simulink model "ConfiguredHevMmVirtualVehicle"  (R2025b)
settings: configuration reference "VehicleVariable" (kept outside this file)
StartFcn:
  | %tic
StopFcn:
  | %toc
model workspace (MAT data in the model file):
  ExtDrvCmdsSwitch = Simulink.Parameter
  ExtDrvCmdsSwitch.Value = 0
  ExtDrvCmdsSwitch.Complexity = 'real'
  ExtDrvCmdsSwitch.Dimensions = [1 1]
  ExtDrvCmdsSwitch.DataType = 'boolean'
  ExtDrvRefSwitch = Simulink.Parameter
  ExtDrvRefSwitch.Value = 0
  ExtDrvRefSwitch.Complexity = 'real'
  ExtDrvRefSwitch.Dimensions = [1 1]
  ExtDrvRefSwitch.DataType = 'boolean'
  ExtEnvSwitch = Simulink.Parameter
  ExtEnvSwitch.Value = 0
  ExtEnvSwitch.Complexity = 'real'
  ExtEnvSwitch.Dimensions = [1 1]
  ExtEnvSwitch.DataType = 'boolean'
  ExtGndSwitch = Simulink.Parameter
  ExtGndSwitch.Value = 0
  ExtGndSwitch.Complexity = 'real'
  ExtGndSwitch.Dimensions = [1 1]
  ExtGndSwitch.DataType = 'boolean'
undefined symbols (not defined in the file or in its folder): AmbTemp, BaroPress, CurvGradRef, CurvRef, DCM, DriverAeroRes, DriverDrivelineRes, DriverInitialGear, DriverPreviewDist, DriverRollRes, DriverShiftTime, DriverTimeConst, DriverTractiveForce, EnvAbsPrs, EnvAirTemp, EnvGrvty, EnvNomFrictionScaling, EnvNominalGrade, EnvScnFrictionMap, EnvScnFrictionMapXBpts, EnvScnFrictionMapYBpts, EnvScnHeightMap, EnvScnHeightMapXBpts, EnvScnHeightMapYBpts, EnvWindVelX, EnvWindVelY, EnvWindVelZ, Gnd, Grade, HazzardCmd, HighBeamCmd, lambda_mux, LeftSignalCmd, LngRef, LowBeamCmd, LtrRef, PhiRef, PlntVehDstCGFrntAxl, PlntVehDstCGRearAxl, PlntVehInitLatPos, PlntVehInitLongPos, PlntVehInitPitchAng, PlntVehInitRollAng, PlntVehInitVertPos, PlntVehInitYawAng, PlntVehMass, PlntVehTrckWdth, PlntVehYawMomentInertia, PlntWhlLdRadiusFrnt, PlntWhlLdRadiusRear, RightSignalCmd, ScnCRRadius, Sim3dSensor, Wind, XRef, YRef, Z
libraries: simulink x28, autolibutils x8, autolibsharedcommon x7, vehdynlibscenariocommon x7, vehdynlibviscommon x4, vehdynlibdriver x2, sim3dgroundtruthsensorlib x2, sim3dlib x2, autolibshared x2, sim3dautolib x2, sl3dlib x1, sharedtransform x1
(part 1 of 6)
settings Model: DataDictionary=VirtualVehicleTemplate.sldd  ModifiedByFormat=The MathWorks, Inc.  SimulationMode=accelerator  ParameterArgumentNames=ExtDrvCmdsSwitch,ExtDrvRefSwitch,ExtEnvSwitch,ExtGndSwitch  Creator=The MathWorks, Inc.  LastModifiedBy=The MathWorks, Inc.
settings ConfigSetRef: SourceName=VehicleVariable

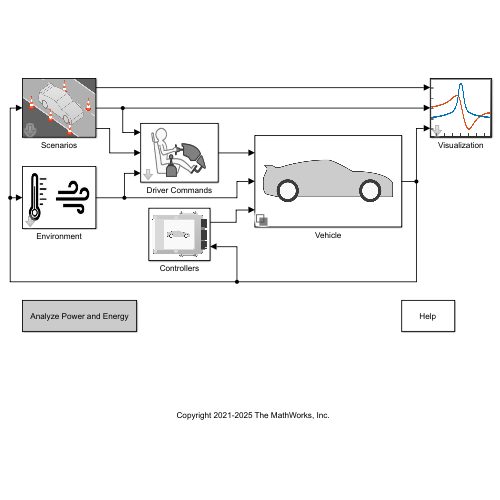
[thumbnail: Simulink's stored preview of the top-level diagram]
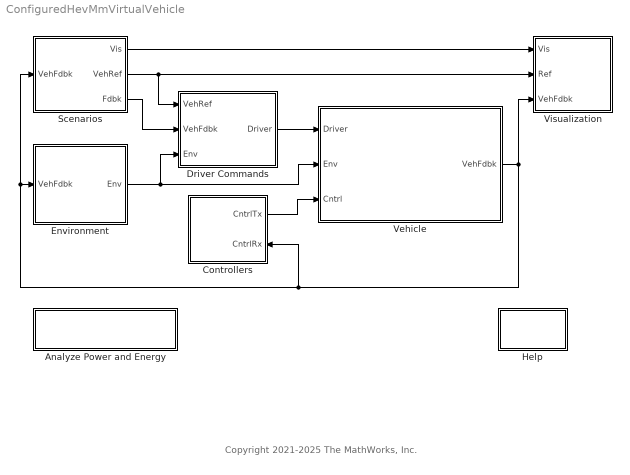
== system ConfiguredHevMmVirtualVehicle ==
  note: Copyright 2021-2025 The MathWorks, Inc.
  Analyze Power and Energy : Subsystem
      settings: OpenFcn=GenerateEnergyReportM2MLX
      mask Display: disp(getString(message('autoblks:autoblkVehMask:powAndEne')))
  Controllers : Subsystem
      settings: PortSchema="{\"entries\":[{\"content\":{\"sides\":[{\"content\":{\"connectorIds\":[]},\"type\":\"ConnectorPlacement.EquallySpacedRectSide\",\"uuid\":\"a925dd9c-6905-4c67-a62c-b22bb69d2bd6\"},{\"content\":{\"connectorIds\":[\"Out1\",\"In1\"],\"side\":\"RIGHT\"},\"type\":\"ConnectorPlacement.EquallySpacedRectSide\",\"uuid\":\"9930ed3e-43a4-46d4-b9ee-7ed64fae32ef\"},{\"content\":{\"connectorIds\":[],\"side\":\"TOP\"},\"type\":\"ConnectorPlacement.EquallySpacedRectSide\",\"uuid\":\"68d2ac4e-de3d-40d3-8b44-059f2a72a6bc\"}]},\"type\":\"ConnectorPlacement.EquallySpacedConnector\",\"uuid\":\"c0be7d07-475b-4046-8bfa-76004f6da9b2\"}],\"packageUris\":[\"http://schema.mathworks.com/mf0/Connector/R2020b\"],\"version\":\"1.0\"}"
      mask Display: image('SystemControllers.png')
  Driver Commands : Subsystem  VariantControl=0  mask(Driver Commands){driverType=Longitudinal Driver}
      mask prompts: driverType "autoblks_reference:autoVirtualRefGen:blkPrm_driverType"
      mask help: autoblks_reference:autoVirtualRefGen:blkDesc_Driver
      mask init:
      | [~]=vdynblksdrvrconfig(gcb);
      mask Help: helpview('autoblks','vvcDriverCommandsHelp')
      mask TypeOptions driverType: autoblks_reference:autoVirtualRefGen:blkCmb_driverType_c1 | autoblks_reference:autoVirtualRefGen:blkCmb_driverType_c2 | autoblks_reference:autoVirtualRefGen:blkCmb_driverType_c3 | autoblks_reference:autoVirtualRefGen:blkCmb_driverType_c4 | autoblks_reference:autoVirtualRefGen:blkCmb_driverType_c5 | autoblks_reference:autoVirtualRefGen:blkCmb_driverType_c6 | autoblks_reference:autoVirtualRefGen:blkCmb_driverType_c7
      mask Callback driverType: [~]=vdynblksdrvrconfig(gcb);
      mask DialogControl driverType Prompt: Vehicle command mode
      mask Display: image('LongitudinalDriver.png');
  Environment : Subsystem  mask(Environment){extEnv=off, extGnd=off}
      mask prompts: extEnv "autoblks_reference:autoVirtualRefGen:blkPrm_extEnv"; extGnd "autoblks_reference:autoVirtualRefGen:blkPrm_extGnd"
      mask help: autoblks_reference:autoVirtualRefGen:blkDesc_Env
      mask Help: helpview('autoblks','vvcEnvironmentHelp')
      mask Callback extEnv: vvcupdateport(gcb,{{'extEnv';'extGnd'},{}},{{'ExtEnv';'ExtGnd'},{}},{{'VVCEnvBUS';'VVCGndSTI4wBUS'},{}});
      mask Callback extGnd: vvcupdateport(gcb,{{'extEnv';'extGnd'},{}},{{'ExtEnv';'ExtGnd'},{}},{{'VVCEnvBUS';'VVCGndSTI4wBUS'},{}});
      mask DialogControl extGroup Prompt: autoblks_reference:autoVirtualRefGen:blkDlg_extGroup
      mask DialogControl extEnv Prompt: Environment
      mask DialogControl extGnd Prompt: Ground
      mask DialogControl EnvButton Prompt: autoblks_reference:autoVirtualRefGen:blkDlg_EnvButton
      mask DialogControl EnvButton Callback: open_system(gcb,'force')
      mask Display: image('Enviroment.png')
  Help : Subsystem
      settings: OpenFcn=helpview('autoblks', 'hybrid_refapp')
      mask Display: disp(getString(message('autoblks:autoblkVehMask:help')))
  Scenarios : Subsystem  mask(Virtual Vehicle Scenario Configuration){extRef=off, extCmd=off}
      mask prompts: extRef "autoblks_reference:autoVirtualRefGen:blkPrm_extRef"; extCmd "autoblks_reference:autoVirtualRefGen:blkPrm_extCmd"
      mask help: autoblks_reference:autoVirtualRefGen:blkDesc_Scene
      mask Help: helpview('autoblks','vvcScenariosHelp')
      mask Callback extRef: vvcupdateport(gcb,{{'extRef';'extCmd'},{}},{{'ExtDrvRef';'ExtDrvCmd'},{}},{{'VVCDrvRefBUS';'VVCDrvCmdBUS'},{}});
      mask Callback extCmd: vvcupdateport(gcb,{{'extRef';'extCmd'},{}},{{'ExtDrvRef';'ExtDrvCmd'},{}},{{'VVCDrvRefBUS';'VVCDrvCmdBUS'},{}});
      mask DialogControl extGroup Prompt: autoblks_reference:autoVirtualRefGen:blkDlg_extGroup
      mask DialogControl extRef Prompt: Driver reference
      mask DialogControl extCmd Prompt: Driver commands
      mask Display: image('vdbslibscen_vvc.png')
  Vehicle : Subsystem  Variant=on  VariantChoicesSpecifier={'ConfiguredSimulinkPlantModel'}  VariantControlMode=label  VariantControl=Vehicle  LabelModeActiveChoice=ConfiguredSimulinkPlantModel
      mask Display: image('PassengerVehicle.png'); % Use "Edit Image" on toolstrip to change.
  Visualization : Subsystem  mask(Visualization){extVehFdbk=off}
      mask prompts: extVehFdbk "autoblks_reference:autoVirtualRefGen:blkPrm_extVehFdbk"
      mask help: autoblks_reference:autoVirtualRefGen:blkDesc_Vis
      mask Help: helpview('autoblks','vvcVisualizationHelp')
      mask Callback extVehFdbk: vvcupdateport(gcb,{{},{'extVehFdbk'}},{{},{'ExtVehFdbk'}},{{},{'VVCVehFdbk'}});
      mask DialogControl extOutGroup Prompt: autoblks_reference:autoVirtualRefGen:blkDlg_extOutGroup
      mask DialogControl extVehFdbk Prompt: Vehicle feedback
      mask DialogControl visButton Prompt: autoblks_reference:autoVirtualRefGen:blkDlg_visButton
      mask DialogControl visButton Callback: open_system(gcb,'force')
      mask Display: image('Visualization.png')
  wires:
  Vehicle/1(VehFdbk) -> Visualization/3(VehFdbk), Controllers/1(CntrlRx), Environment/1(VehFdbk), Scenarios/1(VehFdbk)
  Controllers/1(CntrlTx) -> Vehicle/3(Cntrl)
  Scenarios/2(VehRef) -> Driver Commands/1(VehRef), Visualization/2(Ref)
  Scenarios/3(Fdbk) -> Driver Commands/2(VehFdbk)
  Driver Commands/1(Driver) -> Vehicle/1(Driver)
  Scenarios/1(Vis) -> Visualization/1(Vis)
  Environment/1(Env) -> Driver Commands/3(Env), Vehicle/2(Env)

== system ConfiguredHevMmVirtualVehicle/Analyze Power and Energy ==

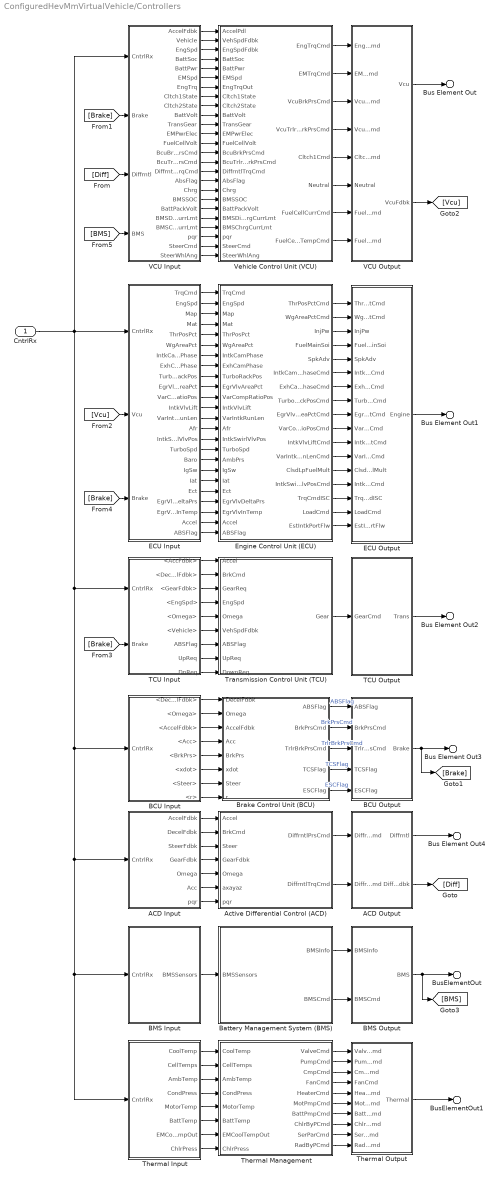
== system ConfiguredHevMmVirtualVehicle/Controllers ==
  CntrlRx : Inport
  ACD Input : Subsystem
  ACD Output : Subsystem
  Active Differential Control (ACD) : Subsystem  Variant=on  VariantChoicesSpecifier={'NoDifferentialControl'}  VariantControlMode=label  LabelModeActiveChoice=NoDifferentialControl
  BCU Input : Subsystem
  BCU Output : Subsystem
  BMS Input : Subsystem
  BMS Output : Subsystem
  Battery Management System (BMS) : Subsystem  Variant=on  VariantChoicesSpecifier={'NoBMS'}  VariantControlMode=label  LabelModeActiveChoice=NoBMS
  Brake Control Unit (BCU) : Subsystem  Variant=on  VariantChoicesSpecifier={'OpenLoopBraking'}  VariantControlMode=label  LabelModeActiveChoice=OpenLoopBraking
  ECU Input : Subsystem
  ECU Output : Subsystem
  Engine Control Unit (ECU) : Subsystem  Variant=on  VariantChoicesSpecifier={'SiEngineController'}  VariantControlMode=label  LabelModeActiveChoice=SiEngineController
  TCU Input : Subsystem
  TCU Output : Subsystem
  Thermal Input : Subsystem
  Thermal Management : Subsystem  Variant=on  VariantChoicesSpecifier={'NoThermalControl'}  VariantControlMode=label  LabelModeActiveChoice=NoThermalControl
  Thermal Output : Subsystem
  Transmission Control Unit (TCU) : Subsystem  Variant=on  VariantChoicesSpecifier={'DriverPassThrough'}  VariantControlMode=label  VariantControl=Variant1  LabelModeActiveChoice=DriverPassThrough
  VCU Input : Subsystem
  VCU Output : Subsystem
  Vehicle Control Unit (VCU) : Subsystem  Variant=on  VariantChoicesSpecifier={'HevMmPowertrainController'}  VariantControlMode=label  LabelModeActiveChoice=HevMmPowertrainController
  Bus Element Out : Outport  PortName=CntrlTx  Element=Vcu
  Bus Element Out1 : Outport  PortName=CntrlTx  Element=Engine
  Bus Element Out2 : Outport  PortName=CntrlTx  Element=Trans
  Bus Element Out3 : Outport  PortName=CntrlTx  Element=Brake
  Bus Element Out4 : Outport  PortName=CntrlTx  Element=Diff
  BusElementOut : Outport  PortName=CntrlTx  Element=BMS
  BusElementOut1 : Outport  PortName=CntrlTx  Element=Thermal
  wires:
  ECU Input/1(TrqCmd) -> Engine Control Unit (ECU)/1(TrqCmd)
  VCU Input/1(AccelFdbk) -> Vehicle Control Unit (VCU)/1(AccelPdl)
  VCU Input/2(Vehicle) -> Vehicle Control Unit (VCU)/2(VehSpdFdbk)
  VCU Input/3(EngSpd) -> Vehicle Control Unit (VCU)/3(EngSpdFdbk)
  VCU Input/4(BattSoc) -> Vehicle Control Unit (VCU)/4(BattSoc)
  VCU Input/5(BattPwr) -> Vehicle Control Unit (VCU)/5(BattPwr)
  VCU Input/6(EMSpd) -> Vehicle Control Unit (VCU)/6(EMSpd)
  VCU Input/7(EngTrq) -> Vehicle Control Unit (VCU)/7(EngTrqOut)
  VCU Input/8(Cltch1State) -> Vehicle Control Unit (VCU)/8(Cltch1State)
  VCU Input/9(Cltch2State) -> Vehicle Control Unit (VCU)/9(Cltch2State)
  VCU Input/10(BattVolt) -> Vehicle Control Unit (VCU)/10(BattVolt)
  VCU Input/11(TransGear) -> Vehicle Control Unit (VCU)/11(TransGear)
  VCU Input/12(EMPwrElec) -> Vehicle Control Unit (VCU)/12(EMPwrElec)
  VCU Input/13(FuelCellVolt) -> Vehicle Control Unit (VCU)/13(FuelCellVolt)
  VCU Input/18(Chrg) -> Vehicle Control Unit (VCU)/18(Chrg)
  VCU Input/17(AbsFlag) -> Vehicle Control Unit (VCU)/17(AbsFlag)
  VCU Input/16(DiffrntlTrqCmd) -> Vehicle Control Unit (VCU)/16(DiffrntlTrqCmd)
  VCU Input/14(BcuBrkPrsCmd) -> Vehicle Control Unit (VCU)/14(BcuBrkPrsCmd)
  ECU Input/2(EngSpd) -> Engine Control Unit (ECU)/2(EngSpd)
  ECU Input/3(Map) -> Engine Control Unit (ECU)/3(Map)
  ECU Input/4(Mat) -> Engine Control Unit (ECU)/4(Mat)
  ECU Input/5(ThrPosPct) -> Engine Control Unit (ECU)/5(ThrPosPct)
  ECU Input/6(WgAreaPct) -> Engine Control Unit (ECU)/6(WgAreaPct)
  ECU Input/7(IntkCamPhase) -> Engine Control Unit (ECU)/7(IntkCamPhase)
  ECU Input/8(ExhCamPhase) -> Engine Control Unit (ECU)/8(ExhCamPhase)
  ECU Input/9(TurboRackPos) -> Engine Control Unit (ECU)/9(TurboRackPos)
  ECU Input/10(EgrVlvAreaPct) -> Engine Control Unit (ECU)/10(EgrVlvAreaPct)
  ECU Input/11(VarCompRatioPos) -> Engine Control Unit (ECU)/11(VarCompRatioPos)
  ECU Input/12(IntkVlvLift) -> Engine Control Unit (ECU)/12(IntkVlvLift)
  ECU Input/13(VarIntkRunLen) -> Engine Control Unit (ECU)/13(VarIntkRunLen)
  ECU Input/14(Afr) -> Engine Control Unit (ECU)/14(Afr)
  ECU Input/15(IntkSwirlVlvPos) -> Engine Control Unit (ECU)/15(IntkSwirlVlvPos)
  ECU Input/16(TurboSpd) -> Engine Control Unit (ECU)/16(TurboSpd)
  ECU Input/17(Baro) -> Engine Control Unit (ECU)/17(AmbPrs)
  ECU Input/18(IgSw) -> Engine Control Unit (ECU)/18(IgSw)
  ECU Input/19(Iat) -> Engine Control Unit (ECU)/19(Iat)
  ECU Input/20(Ect) -> Engine Control Unit (ECU)/20(Ect)
  ECU Input/21(EgrVlvDeltaPrs) -> Engine Control Unit (ECU)/21(EgrVlvDeltaPrs)
  ECU Input/22(EgrVlvInTemp) -> Engine Control Unit (ECU)/22(EgrVlvInTemp)
  TCU Input/8(UpReq) -> Transmission Control Unit (TCU)/8(UpReq)
  TCU Input/1(<AccFdbk>) -> Transmission Control Unit (TCU)/1(Accel)
  TCU Input/2(<DecelFdbk>) -> Transmission Control Unit (TCU)/2(BrkCmd)
  TCU Input/3(<GearFdbk>) -> Transmission Control Unit (TCU)/3(GearReq)
  TCU Input/4(<EngSpd>) -> Transmission Control Unit (TCU)/4(EngSpd)
  TCU Input/5(<Omega>) -> Transmission Control Unit (TCU)/5(Omega)
  TCU Input/6(<Vehicle>) -> Transmission Control Unit (TCU)/6(VehSpdFdbk)
  TCU Input/7(ABSFlag) -> Transmission Control Unit (TCU)/7(ABSFlag)
  TCU Input/9(DnReq) -> Transmission Control Unit (TCU)/9(DownReq)
  ACD Input/1(AccelFdbk) -> Active Differential Control (ACD)/1(Accel)
  ACD Input/2(DecelFdbk) -> Active Differential Control (ACD)/2(BrkCmd)
  ACD Input/3(SteerFdbk) -> Active Differential Control (ACD)/3(Steer)
  ACD Input/4(GearFdbk) -> Active Differential Control (ACD)/4(GearFdbk)
  ACD Input/5(Omega) -> Active Differential Control (ACD)/5(Omega)
  ACD Input/6(Acc) -> Active Differential Control (ACD)/6(axayaz)
  ACD Input/7(pqr) -> Active Differential Control (ACD)/7(pqr)
  Active Differential Control (ACD)/1(DiffrntlPrsCmd) -> ACD Output/1(DiffrntlPrsCmd)
  Active Differential Control (ACD)/2(DiffrntlTrqCmd) -> ACD Output/2(DiffrntlTrqCmd)
  ACD Output/1(Diffrntl) -> Bus Element Out4/1
  Transmission Control Unit (TCU)/1(" Gear") -> TCU Output/1(GearCmd)
  TCU Output/1(Trans) -> Bus Element Out2/1
  Vehicle Control Unit (VCU)/1(EngTrqCmd) -> VCU Output/1(EngTrqCmd)
  Vehicle Control Unit (VCU)/2(EMTrqCmd) -> VCU Output/2(EMTrqCmd)
  Vehicle Control Unit (VCU)/3(VcuBrkPrsCmd) -> VCU Output/3(VcuBrkPrsCmd)
  Vehicle Control Unit (VCU)/5(Cltch1Cmd) -> VCU Output/5(Cltch1Cmd)
  Vehicle Control Unit (VCU)/6(Neutral) -> VCU Output/6(Neutral)
  Vehicle Control Unit (VCU)/7(FuelCellCurrCmd) -> VCU Output/7(FuelCellCurrCmd)
  Vehicle Control Unit (VCU)/8(FuelCellTempCmd) -> VCU Output/8(FuelCellTempCmd)
  BCU Output/1(Brake) -> [Brake], Bus Element Out3/1
  Engine Control Unit (ECU)/1(ThrPosPctCmd) -> ECU Output/1(ThrPosPctCmd)
  Engine Control Unit (ECU)/2(WgAreaPctCmd) -> ECU Output/2(WgAreaPctCmd)
  Engine Control Unit (ECU)/3(InjPw) -> ECU Output/3(InjPw)
  Engine Control Unit (ECU)/4(FuelMainSoi) -> ECU Output/4(FuelMainSoi)
  Engine Control Unit (ECU)/5(SpkAdv) -> ECU Output/5(SpkAdv)
  Engine Control Unit (ECU)/6(IntkCamPhaseCmd) -> ECU Output/6(IntkCamPhaseCmd)
  Engine Control Unit (ECU)/7(ExhCamPhaseCmd) -> ECU Output/7(ExhCamPhaseCmd)
  Engine Control Unit (ECU)/8(TurboRackPosCmd) -> ECU Output/8(TurboRackPosCmd)
  Engine Control Unit (ECU)/9(EgrVlvAreaPctCmd) -> ECU Output/9(EgrVlvAreaPctCmd)
  Engine Control Unit (ECU)/10(VarCompRatioPosCmd) -> ECU Output/10(VarCompRatioPosCmd)
  Engine Control Unit (ECU)/11(IntkVlvLiftCmd) -> ECU Output/11(IntkVlvLiftCmd)
  Engine Control Unit (ECU)/12(VarIntkRunLenCmd) -> ECU Output/12(VarIntkRunLenCmd)
  Engine Control Unit (ECU)/13(ClsdLpFuelMult) -> ECU Output/13(ClsdLpFuelMult)
  Engine Control Unit (ECU)/14(IntkSwirlVlvPosCmd) -> ECU Output/14(IntkSwirlVlvPosCmd)
  Engine Control Unit (ECU)/15(TrqCmdISC) -> ECU Output/15(TrqCmdISC)
  Engine Control Unit (ECU)/16(LoadCmd) -> ECU Output/16(LoadCmd)
  Engine Control Unit (ECU)/17(EstIntkPortFlw) -> ECU Output/17(EstIntkPortFlw)
  ECU Output/1(Engine) -> Bus Element Out1/1
  [Brake] -> VCU Input/2(Brake)
  [Diff] -> VCU Input/3(Diffrntl)
  [Vcu] -> ECU Input/2(Vcu)
  [Brake] -> TCU Input/2(Brake)
  ECU Input/23(Accel) -> Engine Control Unit (ECU)/23(Accel)
  ECU Input/24(ABSFlag) -> Engine Control Unit (ECU)/24(ABSFlag)
  [Brake] -> ECU Input/3(Brake)
  BMS Input/1(BMSSensors) -> Battery Management System (BMS)/1(BMSSensors)
  Battery Management System (BMS)/1(BMSInfo) -> BMS Output/1(BMSInfo)
  Battery Management System (BMS)/2(BMSCmd) -> BMS Output/2(BMSCmd)
  BMS Output/1(BMS) -> BusElementOut/1, [BMS]
  [BMS] -> VCU Input/4(BMS)
  VCU Input/19(BMSSOC) -> Vehicle Control Unit (VCU)/19(BMSSOC)
  VCU Input/20(BattPackVolt) -> Vehicle Control Unit (VCU)/20(BattPackVolt)
  VCU Input/21(BMSDischrgCurrLmt) -> Vehicle Control Unit (VCU)/21(BMSDischrgCurrLmt)
  VCU Input/22(BMSChrgCurrLmt) -> Vehicle Control Unit (VCU)/22(BMSChrgCurrLmt)
  Vehicle Control Unit (VCU)/4(VcuTrlrBrkPrsCmd) -> VCU Output/4(VcuTrlrBrkPrsCmd)
  VCU Input/15(BcuTrlrBrkPrsCmd) -> Vehicle Control Unit (VCU)/15(BcuTrlrBrkPrsCmd)
  VCU Input/23(pqr) -> Vehicle Control Unit (VCU)/23(pqr)
  VCU Input/24(SteerCmd) -> Vehicle Control Unit (VCU)/24(SteerCmd)
  VCU Input/25(SteerWhlAng) -> Vehicle Control Unit (VCU)/25(SteerWhlAng)
  CntrlRx/1 -> VCU Input/1(CntrlRx), ECU Input/1(CntrlRx), TCU Input/1(CntrlRx), BCU Input/1(CntrlRx), ACD Input/1(CntrlRx), Thermal Input/1(CntrlRx), BMS Input/1(CntrlRx)
  VCU Output/1(Vcu) -> Bus Element Out/1
  VCU Output/2(VcuFdbk) -> [Vcu]
  ACD Output/2(DiffrntlFdbk) -> [Diff]
  Thermal Output/1(Thermal) -> BusElementOut1/1
  Brake Control Unit (BCU)/1(ABSFlag) -> BCU Output/1(ABSFlag)  "ABSFlag"
  Brake Control Unit (BCU)/2(BrkPrsCmd) -> BCU Output/2(BrkPrsCmd)  "BrkPrsCmd"
  Brake Control Unit (BCU)/3(TrlrBrkPrsCmd) -> BCU Output/3(TrlrBrkPrsCmd)  "TrlrBrkPrsCmd"
  Brake Control Unit (BCU)/4(TCSFlag) -> BCU Output/4(TCSFlag)  "TCSFlag"
  Brake Control Unit (BCU)/5(ESCFlag) -> BCU Output/5(ESCFlag)  "ESCFlag"
  BCU Input/1(<DecelFdbk>) -> Brake Control Unit (BCU)/1(DecelFdbk)
  BCU Input/2(<Omega>) -> Brake Control Unit (BCU)/2(Omega)
  BCU Input/3(<AccelFdbk>) -> Brake Control Unit (BCU)/3(AccelFdbk)
  BCU Input/4(<Acc>) -> Brake Control Unit (BCU)/4(Acc)
  BCU Input/5(<BrkPrs>) -> Brake Control Unit (BCU)/5(BrkPrs)
  BCU Input/6(<xdot>) -> Brake Control Unit (BCU)/6(xdot)
  BCU Input/7(<Steer>) -> Brake Control Unit (BCU)/7(Steer)
  BCU Input/8(<r>) -> Brake Control Unit (BCU)/8(r)
  Thermal Management/9(SerParCmd) -> Thermal Output/9(SerParCmd)
  Thermal Management/2(PumpCmd) -> Thermal Output/2(PumpCmd)
  Thermal Input/4(CondPress) -> Thermal Management/4(CondPress)
  Thermal Management/6(MotPmpCmd) -> Thermal Output/6(MotPmpCmd)
  Thermal Input/1(CoolTemp) -> Thermal Management/1(CoolTemp)
  Thermal Input/7(EMCoolTempOut) -> Thermal Management/7(EMCoolTempOut)
  Thermal Management/5(HeaterCmd) -> Thermal Output/5(HeaterCmd)
  Thermal Input/5(MotorTemp) -> Thermal Management/5(MotorTemp)
  Thermal Management/1(ValveCmd) -> Thermal Output/1(ValveCmd)
  Thermal Management/3(CmpCmd) -> Thermal Output/3(CmpCmd)
  Thermal Management/7(BattPmpCmd) -> Thermal Output/7(BattPmpCmd)
  Thermal Input/2(CellTemps) -> Thermal Management/2(CellTemps)
  Thermal Input/6(BattTemp) -> Thermal Management/6(BattTemp)
  Thermal Management/4(FanCmd) -> Thermal Output/4(FanCmd)
  Thermal Input/3(AmbTemp) -> Thermal Management/3(AmbTemp)
  Thermal Management/8(ChlrByPCmd) -> Thermal Output/8(ChlrPyPCmd)
  Thermal Management/10(RadByPCmd) -> Thermal Output/10(RadByPCmd)
  Thermal Input/8(ChlrPress) -> Thermal Management/8(ChlrPress)

== system ConfiguredHevMmVirtualVehicle/Driver Commands ==
  VehRef : Inport
  VehFdbk : Inport  Port=2
  Env : Inport  Port=3
  AccelGround : Ground
  BrakeGround : Ground
  Driver Commands : Subsystem  Variant=on  VariantControlMode=label  VariantControl=Variant1  LabelModeActiveChoice=Longitudinal Driver
  GearGround : Ground
  SteerGround : Ground
  Driver : Outport  VectorParamsAs1DForOutWhenUnconnected=off
  wires:
  Env/1 -> Driver Commands/3(Env)
  Driver Commands/1(" Driver") -> Driver/1
  VehFdbk/1 -> Driver Commands/2(VehFdbk)
  VehRef/1 -> Driver Commands/1(VehRef)
  SteerGround/1 -> Driver Commands/4(SteerCmd)
  AccelGround/1 -> Driver Commands/5(AccelCmd)
  BrakeGround/1 -> Driver Commands/6(BrakeCmd)
  GearGround/1 -> Driver Commands/7(GearCmd)

== system ConfiguredHevMmVirtualVehicle/Environment ==
  note: The Ground Feedback variant subsystem is automatically enabled/disabled according to the 3D Engine settings found in the Reference Generator.
      | Manually overriding this variant may result in initialization errors.
  In Bus Element8 : Inport  PortName=VehFdbk  Element=Body.InertFrm
  In Bus Element1 : Inport  PortName=VehFdbk  Element=Body.InertFrm.Cg.Disp
  BusElementIn3 : Inport  PortName=VehFdbk  Element=FrntWheels.Wheels.z
  BusElementIn1 : Inport  PortName=VehFdbk  Element=FrntWheels.Wheels.Omega
  BusElementIn : Inport  PortName=VehFdbk  Element=FrntSuspension.FrntSuspChassis.Whl.Ang
  BusElementIn2 : Inport  PortName=VehFdbk  Element=RearWheels.Wheels.z
  BusElementIn4 : Inport  PortName=VehFdbk  Element=RearWheels.Wheels.Omega
  BusElementIn5 : Inport  PortName=VehFdbk  Element=RearSuspension.RearSuspChassis.Whl.Ang
  Baro_Pa : Constant  Value=EnvAbsPrs  SampleTime=0
  Bus Creator : BusCreator  Inputs=3
  Bus Creator2 : BusCreator  Inputs=4
  Bus Creator3 : BusCreator  Inputs=3
  Bus to Vector : BusToVector
  Bus to Vector1 : BusToVector
  Constant3 : Constant  Value=EnvWindVelX  SampleTime=0
  Constant4 : Constant  Value=EnvWindVelY  SampleTime=0
  Constant5 : Constant  Value=EnvWindVelZ  SampleTime=0
  Demux1 : Demux
  ExtEnvConstant : Constant  Value=0  OutDataTypeStr=Bus: VVCEnvBUS
  ExtGndConstant : Constant  Value=0  OutDataTypeStr=Bus: VVCGndSTI4wBUS
  Ground Feedback : Subsystem  Variant=on  VariantControlMode=label  LabelModeActiveChoice=0
  Signal Specification1 : SignalSpecification  Unit=1
  Subsystem : Subsystem
  Temp_degK : Constant  Value=EnvAirTemp  SampleTime=0
  Varying Friction : Subsystem  Variant=on  VariantControlMode=label  VariantControl=Choice  LabelModeActiveChoice=0
  Vector Concatenate : Concatenate  NumInputs=3
  Vector Concatenate1 : Concatenate
  Vector Concatenate2 : Concatenate
  Vector Concatenate3 : Concatenate  Mode=Multidimensional array  ConcatenateDimension=2
  Env : Outport  VectorParamsAs1DForOutWhenUnconnected=off
  wires:
  Constant5/1 -> Vector Concatenate/3  "Z"
  Constant3/1 -> Vector Concatenate/1  "X"
  Constant4/1 -> Vector Concatenate/2  "Y"
  In Bus Element1/1 -> Varying Friction/2(Cg)
  BusElementIn3/1 -> Vector Concatenate1/1  "z"
  BusElementIn1/1 -> Bus to Vector/1  "Omega"
  BusElementIn/1 -> Vector Concatenate3/1  "WhlAng"
  Bus Creator/1 -> Ground Feedback/1(WheelFdbk)  "WheelFdbk"
  Temp_degK/1 -> Subsystem/3(AmbTemp)
  Baro_Pa/1 -> Subsystem/4(BaroPress)
  Vector Concatenate/1 -> Subsystem/5(Wind)
  Bus Creator3/1 -> Subsystem/6(InGnd)
  Subsystem/1(Env) -> Env/1
  BusElementIn2/1 -> Vector Concatenate1/2  "z"
  BusElementIn5/1 -> Vector Concatenate3/2  "WhlAng"
  BusElementIn4/1 -> Bus to Vector1/1  "Omega"
  Vector Concatenate1/1 -> Bus Creator/1  "z"
  Vector Concatenate2/1 -> Bus Creator/2  "Omega"
  Vector Concatenate3/1 -> Bus Creator/3  "WhlAng"
  Bus to Vector/1 -> Vector Concatenate2/1
  Bus to Vector1/1 -> Vector Concatenate2/2
  Ground Feedback/1(Z) -> Bus Creator3/1  "z"
  Demux1/2 -> Bus Creator2/2  "mu_FR"
  Demux1/4 -> Bus Creator2/4  "mu_RR"
  Varying Friction/1(FricCoeffLambda) -> Signal Specification1/1
  Ground Feedback/2(DCM) -> Bus Creator3/2  "DCM"
  Bus Creator2/1 -> Bus Creator3/3  "mu"
  Demux1/1 -> Bus Creator2/1  "mu_FL"
  Demux1/3 -> Bus Creator2/3  "mu_RL"
  Signal Specification1/1 -> Demux1/1
  In Bus Element8/1 -> Ground Feedback/2(InertFrm), Varying Friction/1(InertFrm)
  ExtGndConstant/1 -> Subsystem/2(ExtGnd)
  ExtEnvConstant/1 -> Subsystem/1(ExtEnv)

== system ConfiguredHevMmVirtualVehicle/Help ==

== system ConfiguredHevMmVirtualVehicle/Scenarios ==
  VehFdbk : Inport
  Coordinate Systems : Subsystem  Variant=on  VariantControlMode=label  VariantControl=Choice  LabelModeActiveChoice=ISO 8855 (Z-up)1
  ExtDrvCmdConstant : Constant  Value=0  OutDataTypeStr=Bus: VVCDrvCmdBUS
  ExtDrvRefConstant : Constant  Value=0  OutDataTypeStr=Bus: VVCDrvRefBUS
  Reference Generator : Subsystem  Variant=on  VariantControlMode=label  LabelModeActiveChoice=Drive Cycle
  Reference Routing : Subsystem
  Vis : Outport
  VehRef : Outport  Port=2
  Fdbk : Outport  Port=3
  wires:
  Reference Routing/1(VehRef) -> VehRef/1
  Coordinate Systems/1(ExtDrvRef) -> Reference Routing/1(ExtDrvRef)
  Coordinate Systems/2(ExtDrvCmd) -> Reference Routing/2(ExtDrvCmds)
  VehFdbk/1 -> Reference Generator/1("VehFdbk ")
  Reference Generator/2(DrvCmd) -> Reference Routing/4(DrvCmd)
  Reference Generator/4(" Fdbk") -> Fdbk/1
  Reference Generator/1(DrvRef) -> Reference Routing/3(DrvRef)
  Reference Generator/3(" Vis") -> Vis/1
  ExtDrvCmdConstant/1 -> Coordinate Systems/2(ExtDrvCmdIn)
  ExtDrvRefConstant/1 -> Coordinate Systems/1(ExtDrvRefIn)

== system ConfiguredHevMmVirtualVehicle/Vehicle ==
  Driver : Inport
  Env : Inport  Port=2
  Cntrl : Inport  Port=3
  ConfiguredSimulinkPlantModel : Subsystem  VariantControl=ConfiguredSimulinkPlantModel  ReferencedSubsystem=ConfiguredSimulinkPlantModel
  VehFdbk : Outport

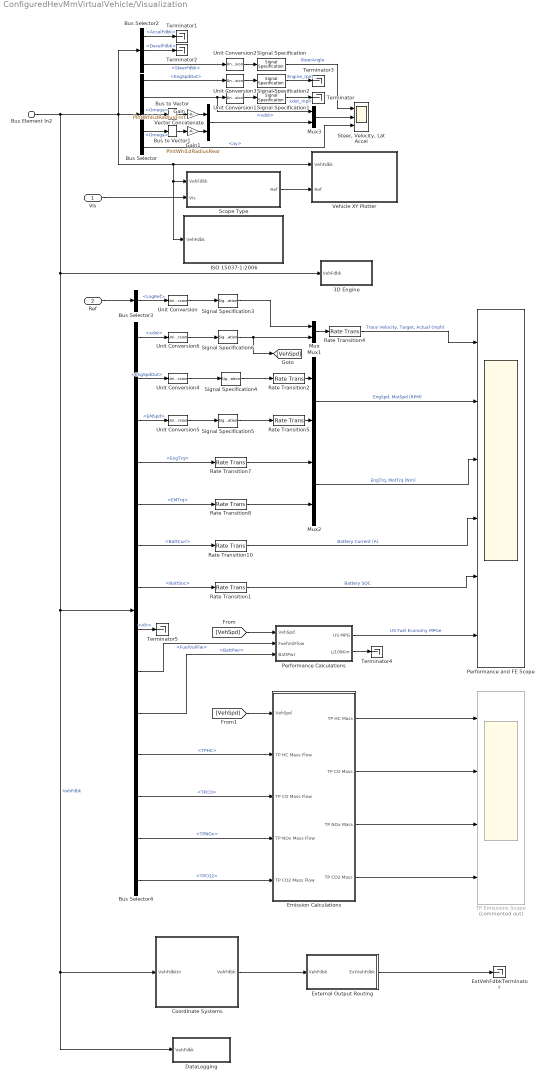
== system ConfiguredHevMmVirtualVehicle/Visualization ==
  Vis : Inport
  Ref : Inport  Port=2
  Bus Element In2 : Inport  Port=3  PortName=VehFdbk
  3D Engine : Subsystem  Variant=on  VariantControlMode=label  LabelModeActiveChoice=NoEngine3D
  Bus Selector : BusSelector  OutputSignals=Engine.EngSpdOut,Body.BdyFrm.Cg.Vel.xdot,FrntWheels.Wheels.Omega,RearWheels.Wheels.Omega,Body.BdyFrm.Cg.Acc.ay
  Bus Selector2 : BusSelector  OutputSignals=Driver.AccelFdbk,Driver.DecelFdbk,Driver.SteerFdbk
  Bus Selector3 : BusSelector  OutputSignals=DrvRef.LngRef
  Bus Selector4 : BusSelector  OutputSignals=Body.BdyFrm.Cg.Vel.xdot,Engine.EngSpdOut,EM.EMSpd,Engine.EngTrq,EM.EMTrq,Battery.BattInfo.BattCurr,Battery.BattInfo.BattSoc,Engine.Afr,Engine.FuelVolFlw,Battery.BattInfo.BattPwr,Engine.TPHC,Engine.TPCO,Engine.TPNOx,Engine.TPCO2
  Bus to Vector : BusToVector
  Bus to Vector1 : BusToVector
  Coordinate Systems : Subsystem  Variant=on  VariantControlMode=label  VariantControl=Choice  LabelModeActiveChoice=ISO 8855 (Z-up)1
  DataLogging : Subsystem
  Emission Calculations : Subsystem
  ExtVehFdbkTerminator : Terminator
  External Output Routing : Subsystem
  Gain : Gain  Gain=PlntWhlLdRadiusFrnt
  Gain1 : Gain  Gain=PlntWhlLdRadiusRear
  ISO 15037-1:2006 : Subsystem  StopFcn=|  Variant=on  VariantControlMode=label  LabelModeActiveChoice=0  mask(ISO 15037-1:2006){Measurement=Disabled}
      | switch get_param(gcb,'Measurement')
      |        case 'Enabled'
      |        VDBSmldatxfolder=[matlabroot '\toolbox\vdynblks\vdynsolution\mldatx'];
      |        Simulink.sdi.loadView([VDBSmldatxfolder filesep 'ISO15037_1_2006E.mldatx']);
      |        Simulink.sdi.view;
      | end
      mask prompts: Measurement "ISO Measurements"
      mask help: Enables display of ISO 15037-1:2006 standard measurement signals in the Simulation Data Inspector.
      mask init:
      | v=ver;
      | isVDBSInstalled=dig.isProductInstalled('Vehicle Dynamics Blockset');
      | maskObj=Simulink.Mask.get(gcb);
      | parameterObj=maskObj.getParameter('Measurement');
      | 
      |     if isVDBSInstalled
      |     
      |         parameterObj.Enabled='on';
      |     
      |         switch get_param(gcb,'Measurement')
      |             case 'Disabled'
      |                 set_param(gcb,'OverrideUsingVariant','0')
      |             case 'Enabled'
      |                set_param(gcb,'OverrideUsingVariant','1')
      |             otherwise
      |                set_param(gcb,'OverrideUsingVariant','0')
      |         end
      |         
      |     else
      |        
      |        parameterObj.Enabled='on'; 
      |        set_param(gcb,'OverrideUsingVariant','0');
      |        parameterObj.Enabled='off';
      |        
      |     end
      settings: AttributesFormatString=%<Measurement>
      mask Help: eval('vdynblkshelp(''iso15037'')');
      mask TypeOptions Measurement: Enabled | Disabled
      mask Callback Measurement:
      | switch get_param(gcb,'Measurement')
      |     case 'Disabled'
      |         set_param(gcb,'OverrideUsingVariant','0')
      |     case 'Enabled'
      |        set_param(gcb,'OverrideUsingVariant','1')
      |     otherwise
      |        set_param(gcb,'OverrideUsingVariant','0')
      | end
      mask Display: disp('ISO 15037-1:2006')
  Mux{,1..3} (4 alike) : Mux  Inputs=2
  Performance Calculations : Subsystem
  Performance and FE Scope : Scope  NumInputPorts=6
      settings: SampleTime=0.1  ActiveDisplayYMinimum=-7.10525  ActiveDisplayYMaximum=63.78947
  Rate Transition{1..2,4..5,7..8,10} (7 alike) : RateTransition  Deterministic=off
  Scope Type : Subsystem  Variant=on  VariantControlMode=label  VariantControl=Variant1  LabelModeActiveChoice=0
  Signal Specification : SignalSpecification  Unit=deg
  Signal Specification1 : SignalSpecification  Unit=mph
  Signal Specification2 : SignalSpecification  Unit=rpm
  Signal Specification3 : SignalSpecification  Unit=mph
  Signal Specification4 : SignalSpecification  Unit=rpm
  Signal Specification5 : SignalSpecification  Unit=rpm
  Signal Specification6 : SignalSpecification  Unit=mph
  "Steer, Velocity, Lat Accel" : Scope  NumInputPorts=3
      settings: ActiveDisplayYMinimum=-4.93239  ActiveDisplayYMaximum=44.39148
  TP Emissions Scope : Scope  Commented=on  NumInputPorts=4
      settings: SampleTime=0.1  ActiveDisplayYMinimum=-0.1021  ActiveDisplayYMaximum=0.91889  DataLoggingVariableName=ScopeData2
  Terminator{,1..5} (6 alike) : Terminator
  Unit Conversion{,1..6} (7 alike) : UnitConversion
  Vector Concatenate : Concatenate
  Vehicle XY Plotter : Subsystem  Variant=on  VariantControlMode=label  VariantControl=Variant1  LabelModeActiveChoice=2
  wires:
  Signal Specification/1 -> "Steer, Velocity, Lat Accel"/1  "SteerAngle"
  Unit Conversion2/1 -> Signal Specification/1
  Vis/1 -> Scope Type/2("Vis ")
  Scope Type/1(" Ref") -> Vehicle XY Plotter/2("Ref ")
  Bus Selector/5 -> "Steer, Velocity, Lat Accel"/3  "<ay>"
  Bus Element In2/1 -> 3D Engine/1(VehFdbk), Bus Selector4/1, DataLogging/1(VehFdbk), Coordinate Systems/1(VehFdbkIn), ISO 15037-1:2006/1(VehFdbk), Scope Type/1("VehFdbk "), Vehicle XY Plotter/1("VehFdbk "), Bus Selector/1, Bus Selector2/1  "VehFdbk"
  Bus Selector/2 -> Mux3/1, Unit Conversion1/1  "<xdot>"
  Bus Selector2/1 -> Terminator1/1  "<AccelFdbk>"
  Bus Selector2/2 -> Terminator2/1  "<DecelFdbk>"
  Bus Selector2/3 -> Unit Conversion2/1  "<SteerFdbk>"
  Rate Transition1/1 -> Performance and FE Scope/5  "Battery SOC"
  Rate Transition2/1 -> Mux1/1
  Signal Specification6/1 -> [VehSpd], Mux/2
  Emission Calculations/4(TP CO2 Mass) -> TP Emissions Scope/4
  Bus Selector4/7 -> Rate Transition1/1  "<BattSoc>"
  Bus Selector4/11 -> Emission Calculations/2(TP HC Mass Flow)  "<TPHC>"
  Bus Selector4/10 -> Performance Calculations/3(BattPwr)  "<BattPwr>"
  Mux/1 -> Rate Transition4/1
  Emission Calculations/2(TP CO Mass) -> TP Emissions Scope/2
  Bus Selector4/12 -> Emission Calculations/3(TP CO Mass Flow)  "<TPCO>"
  Bus Selector4/14 -> Emission Calculations/5(TP CO2 Mass Flow)  "<TPCO2>"
  Bus Selector4/2 -> Unit Conversion4/1  "<EngSpdOut>"
  Performance Calculations/1(US MPG) -> Performance and FE Scope/6  "US Fuel Economy MPGe"
  Bus Selector4/13 -> Emission Calculations/4(TP NOx Mass Flow)  "<TPNOx>"
  Bus Selector4/6 -> Rate Transition10/1  "<BattCurr>"
  Signal Specification5/1 -> Rate Transition5/1
  Rate Transition10/1 -> Performance and FE Scope/4  "Battery Current (A)"
  Signal Specification3/1 -> Mux/1
  Rate Transition5/1 -> Mux1/2
  Rate Transition8/1 -> Mux2/2
  Emission Calculations/3(TP NOx Mass) -> TP Emissions Scope/3
  Rate Transition4/1 -> Performance and FE Scope/1  "Trace Velocity, Target, Actual (mph)"
  Emission Calculations/1(TP HC Mass) -> TP Emissions Scope/1
  Bus Selector4/5 -> Rate Transition8/1  "<EMTrq>"
  Rate Transition7/1 -> Mux2/1
  Mux2/1 -> Performance and FE Scope/3  "EngTrq, MotTrq (Nm)"
  Bus Selector4/8 -> Terminator5/1  "<Afr>"
  Bus Selector4/4 -> Rate Transition7/1  "<EngTrq>"
  Bus Selector4/9 -> Performance Calculations/2(FuelVolFlow)  "<FuelVolFlw>"
  Mux1/1 -> Performance and FE Scope/2  "EngSpd, MotSpd (RPM)"
  Performance Calculations/2(L/100Km) -> Terminator4/1
  Signal Specification4/1 -> Rate Transition2/1
  Ref/1 -> Bus Selector3/1
  Unit Conversion1/1 -> Signal Specification1/1
  Unit Conversion3/1 -> Signal Specification2/1
  Bus Selector/1 -> Unit Conversion3/1  "<EngSpdOut>"
  Signal Specification2/1 -> Terminator3/1  "Engine_rpm"
  Signal Specification1/1 -> Terminator/1  "xdot_mph"
  Unit Conversion/1 -> Signal Specification3/1
  Unit Conversion4/1 -> Signal Specification4/1
  Bus Selector4/3 -> Unit Conversion5/1  "<EMSpd>"
  Unit Conversion5/1 -> Signal Specification5/1
  Bus Selector3/1 -> Unit Conversion/1  "<LngRef>"
  Unit Conversion6/1 -> Signal Specification6/1
  Bus Selector4/1 -> Unit Conversion6/1  "<xdot>"
  [VehSpd] -> Performance Calculations/1(VehSpd)
  [VehSpd] -> Emission Calculations/1(VehSpd)
  Vector Concatenate/1 -> Mux3/2
  Mux3/1 -> "Steer, Velocity, Lat Accel"/2
  Coordinate Systems/1(VehFdbk) -> External Output Routing/1(VehFdbk)
  Bus Selector/3 -> Bus to Vector/1  "<Omega>"
  Bus Selector/4 -> Bus to Vector1/1  "<Omega>"
  Bus to Vector/1 -> Gain/1
  Bus to Vector1/1 -> Gain1/1
  Gain/1 -> Vector Concatenate/1
  Gain1/1 -> Vector Concatenate/2
  External Output Routing/1(ExtVehFdbk) -> ExtVehFdbkTerminator/1

== system ConfiguredHevMmVirtualVehicle/Controllers/ACD Input ==
  CntrlRx : Inport
  Bus Selector3 : BusSelector  OutputSignals=Driver.AccelFdbk,Driver.DecelFdbk,Driver.SteerFdbk,Driver.GearFdbk,FrntWheels.Wheels.Omega,RearWheels.Wheels.Omega,IMU.Acc,IMU.pqr
  Bus to Vector : BusToVector
  Bus to Vector1 : BusToVector
  Rate Transition{1..7} (7 alike) : RateTransition  Deterministic=off
  Vector Concatenate : Concatenate
  AccelFdbk : Outport
  DecelFdbk : Outport  Port=2
  SteerFdbk : Outport  Port=3
  GearFdbk : Outport  Port=4
  Omega : Outport  Port=5
  Acc : Outport  Port=6
  pqr : Outport  Port=7
  wires:
  Bus Selector3/8 -> Rate Transition7/1  "<pqr>"
  Bus Selector3/3 -> Rate Transition2/1  "<SteerFdbk>"
  Bus Selector3/1 -> Rate Transition5/1  "<AccelFdbk>"
  Bus Selector3/7 -> Rate Transition6/1  "<Acc>"
  Bus Selector3/2 -> Rate Transition1/1  "<DecelFdbk>"
  Bus Selector3/4 -> Rate Transition3/1  "<GearFdbk>"
  Vector Concatenate/1 -> Rate Transition4/1
  CntrlRx/1 -> Bus Selector3/1
  Rate Transition5/1 -> AccelFdbk/1
  Rate Transition1/1 -> DecelFdbk/1
  Rate Transition2/1 -> SteerFdbk/1
  Rate Transition3/1 -> GearFdbk/1
  Rate Transition4/1 -> Omega/1
  Rate Transition6/1 -> Acc/1
  Rate Transition7/1 -> pqr/1
  Bus Selector3/5 -> Bus to Vector/1  "<Omega>"
  Bus Selector3/6 -> Bus to Vector1/1  "<Omega>"
  Bus to Vector/1 -> Vector Concatenate/1
  Bus to Vector1/1 -> Vector Concatenate/2

== system ConfiguredHevMmVirtualVehicle/Controllers/ACD Output ==
  DiffrntlPrsCmd : Inport
  DiffrntlTrqCmd : Inport  Port=2
  First Order Hold : FirstOrderHold  ErrorTolerance=inf
  First Order Hold1 : FirstOrderHold  ErrorTolerance=inf
  Out Bus Element : Outport  PortName=Diffrntl  Element=DiffrntlPrsCmd
  Out Bus Element1 : Outport  PortName=Diffrntl  Element=DiffrntlTrqCmd
  Out Bus Element2 : Outport  Port=2  PortName=DiffrntlFdbk  Element=DiffrntlPrsCmd
  Out Bus Element3 : Outport  Port=2  PortName=DiffrntlFdbk  Element=DiffrntlTrqCmd
  wires:
  DiffrntlPrsCmd/1 -> Out Bus Element2/1, First Order Hold/1  "DiffrntlPrsCmd"
  DiffrntlTrqCmd/1 -> Out Bus Element3/1, First Order Hold1/1  "DiffrntlTrqCmd"
  First Order Hold/1 -> Out Bus Element/1
  First Order Hold1/1 -> Out Bus Element1/1

== system ConfiguredHevMmVirtualVehicle/Controllers/Active Differential Control (ACD) ==
  note: 1) Add Subsystem or Model blocks as valid variant choices.
      | 2) You cannot connect blocks at this level. At simulation, connectivity is automatically
      | determined, based on the active variant and port name matching.
  Accel : Inport  PortDimensions=1
  BrkCmd : Inport  Port=2  PortDimensions=1
  Steer : Inport  Port=3
  GearFdbk : Inport  Port=4
  Omega : Inport  Port=5  Unit=rad/s  PortDimensions=4
  axayaz : Inport  Port=6
  pqr : Inport  Port=7
  NoDifferentialControl : ModelReference  ModelNameDialog=NoDifferentialControl  SimulationMode=Normal  VariantControl=NoDifferentialControl  ModelReferenceVersion=3.0
  DiffrntlPrsCmd : Outport  VectorParamsAs1DForOutWhenUnconnected=off
  DiffrntlTrqCmd : Outport  Port=2  VectorParamsAs1DForOutWhenUnconnected=off

== system ConfiguredHevMmVirtualVehicle/Controllers/BCU Input ==
  CntrlRx : Inport
  Add : Sum
  Bus Selector : BusSelector  OutputSignals=Driver.DecelFdbk,FrntWheels.Wheels.Omega,RearWheels.Wheels.Omega,Body.BdyFrm.Cg.Acc.xddot,Driver.AccelFdbk,FrntWheels.Wheels.BrkPrs,RearWheels.Wheels.BrkPrs,Body.BdyFrm.Cg.Vel.xdot,Steering.Front.WhlAng.FL,Steering.Front.WhlAng.FR,Body.BdyFrm.Cg.AngVel.r
  Bus to Vector : BusToVector
  Bus to Vector1 : BusToVector
  Gain : Gain  Gain=0.5
  Rate Transition{1..8} (8 alike) : RateTransition  Deterministic=off
  Vector Concatenate : Concatenate
  Vector Concatenate1 : Concatenate
  <DecelFdbk> : Outport
  <Omega> : Outport  Port=2
  <AccelFdbk> : Outport  Port=3
  <Acc> : Outport  Port=4
  <BrkPrs> : Outport  Port=5
  <xdot> : Outport  Port=6
  <Steer> : Outport  Port=7
  <r> : Outport  Port=8
  wires:
  Vector Concatenate1/1 -> Rate Transition4/1
  Vector Concatenate/1 -> Rate Transition1/1
  CntrlRx/1 -> Bus Selector/1
  Bus Selector/1 -> Rate Transition5/1  "<DecelFdbk>"
  Bus Selector/4 -> Rate Transition2/1  "<xddot>"
  Rate Transition5/1 -> <DecelFdbk>/1
  Rate Transition1/1 -> <Omega>/1
  Rate Transition2/1 -> <Acc>/1
  Rate Transition3/1 -> <AccelFdbk>/1
  Rate Transition4/1 -> <BrkPrs>/1
  Bus Selector/3 -> Bus to Vector1/1  "<Omega>"
  Bus Selector/2 -> Bus to Vector/1  "<Omega>"
  Bus Selector/6 -> Vector Concatenate1/1  "<BrkPrs>"
  Bus Selector/7 -> Vector Concatenate1/2  "<BrkPrs>"
  Bus to Vector/1 -> Vector Concatenate/1
  Bus to Vector1/1 -> Vector Concatenate/2
  Bus Selector/5 -> Rate Transition3/1  "<AccelFdbk>"
  Bus Selector/8 -> Rate Transition6/1  "<xdot>"
  Bus Selector/11 -> Rate Transition8/1  "<r>"
  Rate Transition8/1 -> <r>/1
  Rate Transition6/1 -> <xdot>/1
  Bus Selector/9 -> Add/1  "<FL>"
  Bus Selector/10 -> Add/2  "<FR>"
  Add/1 -> Gain/1
  Gain/1 -> Rate Transition7/1
  Rate Transition7/1 -> <Steer>/1

== system ConfiguredHevMmVirtualVehicle/Controllers/BCU Output ==
  ABSFlag : Inport
  BrkPrsCmd : Inport  Port=2
  TrlrBrkPrsCmd : Inport  Port=3
  TCSFlag : Inport  Port=4
  ESCFlag : Inport  Port=5
  Bus Creator2 : BusCreator  Inputs=5
  Brake : Outport
  wires:
  ABSFlag/1 -> Bus Creator2/1
  Bus Creator2/1 -> Brake/1  "Brake"
  BrkPrsCmd/1 -> Bus Creator2/2
  TrlrBrkPrsCmd/1 -> Bus Creator2/3
  ESCFlag/1 -> Bus Creator2/5
  TCSFlag/1 -> Bus Creator2/4

== system ConfiguredHevMmVirtualVehicle/Controllers/BMS Input ==
  CntrlRx : Inport
  Bus Selector3 : BusSelector  OutputSignals=Battery.BMSSensors
  Rate Transition : RateTransition
  BMSSensors : Outport
  wires:
  CntrlRx/1 -> Bus Selector3/1
  Bus Selector3/1 -> Rate Transition/1  "<BMSSensors>"
  Rate Transition/1 -> BMSSensors/1  "BMSSensors"

== system ConfiguredHevMmVirtualVehicle/Controllers/BMS Output ==
  BMSInfo : Inport
  BMSCmd : Inport  Port=2
  Bus Creator4 : BusCreator  Inputs=2
  BMS : Outport
  wires:
  BMSCmd/1 -> Bus Creator4/2  "BMSCmd"
  Bus Creator4/1 -> BMS/1  "BMS"
  BMSInfo/1 -> Bus Creator4/1  "BMSInfo"

== system ConfiguredHevMmVirtualVehicle/Controllers/Battery Management System (BMS) ==
  BMSSensors : Inport
  NoBMS : ModelReference  ModelNameDialog=NoBMS  SimulationMode=Normal  VariantControl=NoBMS  ModelReferenceVersion=3.0
  BMSInfo : Outport
  BMSCmd : Outport  Port=2

== system ConfiguredHevMmVirtualVehicle/Controllers/Brake Control Unit (BCU) ==
  note: 1) Add Subsystem or Model blocks as valid variant choices.
      | 2) You cannot connect blocks at this level. At simulation, connectivity is automatically
      | determined, based on the active variant and port name matching.
  DecelFdbk : Inport
  Omega : Inport  Port=2
  AccelFdbk : Inport  Port=3
  Acc : Inport  Port=4
  BrkPrs : Inport  Port=5
  xdot : Inport  Port=6
  Steer : Inport  Port=7
  r : Inport  Port=8
  OpenLoopBraking : ModelReference  ModelNameDialog=OpenLoopBraking  SimulationMode=Normal  VariantControl=OpenLoopBraking  ModelReferenceVersion=7.0
  ABSFlag : Outport  VectorParamsAs1DForOutWhenUnconnected=off
  BrkPrsCmd : Outport  Port=2  VectorParamsAs1DForOutWhenUnconnected=off
  TrlrBrkPrsCmd : Outport  Port=3  VectorParamsAs1DForOutWhenUnconnected=off
  TCSFlag : Outport  Port=4  VectorParamsAs1DForOutWhenUnconnected=off
  ESCFlag : Outport  Port=5  VectorParamsAs1DForOutWhenUnconnected=off

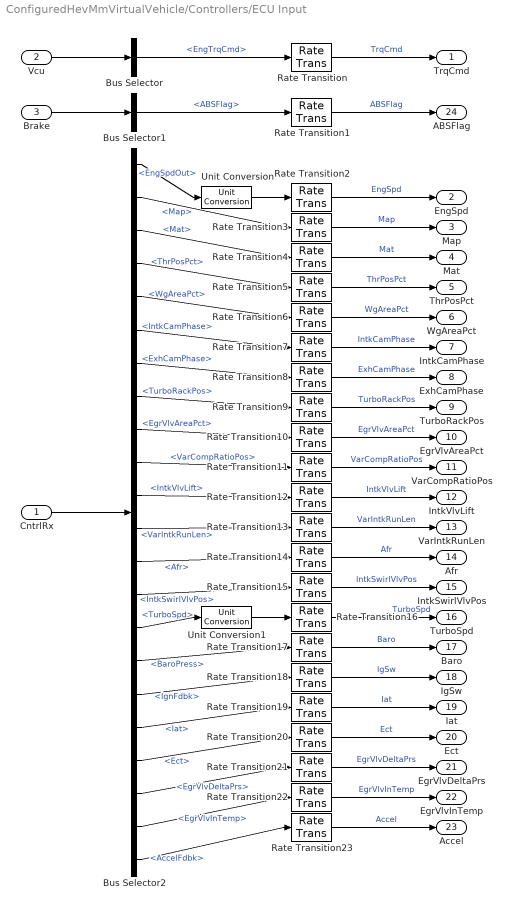
== system ConfiguredHevMmVirtualVehicle/Controllers/ECU Input ==
  CntrlRx : Inport
  Vcu : Inport  Port=2
  Brake : Inport  Port=3
  Bus Selector : BusSelector  OutputSignals=EngTrqCmd
  Bus Selector1 : BusSelector  OutputSignals=ABSFlag
  Bus Selector2 : BusSelector  OutputSignals=Engine.EngSpdOut,Engine.Map,Engine.Mat,Engine.ThrPosPct,Engine.WgAreaPct,Engine.IntkCamPhase,Engine.ExhCamPhase,Engine.TurboRackPos,Engine.EgrVlvAreaPct,Engine.VarCompRatioPos,Engine.IntkVlvLift,Engine.VarIntkRunLen,Engine.Afr,Engine.IntkSwirlVlvPos,Engine.TurboSpd,Env.BaroPress,Driver.IgnFdbk,Engine.Iat,Engine.Ect,Engine.EgrVlvDeltaPrs,Engine.EgrVlvInTemp,Driver.AccelFdbk
  Rate Transition{,1..23} (24 alike) : RateTransition  Deterministic=off
  Unit Conversion : UnitConversion
  Unit Conversion1 : UnitConversion
  TrqCmd : Outport
  EngSpd : Outport  Port=2
  Map : Outport  Port=3
  Mat : Outport  Port=4
  ThrPosPct : Outport  Port=5
  WgAreaPct : Outport  Port=6
  IntkCamPhase : Outport  Port=7
  ExhCamPhase : Outport  Port=8
  TurboRackPos : Outport  Port=9
  EgrVlvAreaPct : Outport  Port=10
  VarCompRatioPos : Outport  Port=11
  IntkVlvLift : Outport  Port=12
  VarIntkRunLen : Outport  Port=13
  Afr : Outport  Port=14
  IntkSwirlVlvPos : Outport  Port=15
  TurboSpd : Outport  Port=16
  Baro : Outport  Port=17
  IgSw : Outport  Port=18
  Iat : Outport  Port=19
  Ect : Outport  Port=20
  EgrVlvDeltaPrs : Outport  Port=21
  EgrVlvInTemp : Outport  Port=22
  Accel : Outport  Port=23
  ABSFlag : Outport  Port=24
  wires:
  Bus Selector2/13 -> Rate Transition14/1  "<Afr>"
  Bus Selector2/1 -> Unit Conversion/1  "<EngSpdOut>"
  Bus Selector2/21 -> Rate Transition22/1  "<EgrVlvInTemp>"
  Bus Selector2/19 -> Rate Transition20/1  "<Ect>"
  Bus Selector2/9 -> Rate Transition10/1  "<EgrVlvAreaPct>"
  Bus Selector2/15 -> Unit Conversion1/1  "<TurboSpd>"
  Bus Selector2/17 -> Rate Transition18/1  "<IgnFdbk>"
  Bus Selector2/16 -> Rate Transition17/1  "<BaroPress>"
  Bus Selector2/2 -> Rate Transition3/1  "<Map>"
  Bus Selector2/18 -> Rate Transition19/1  "<Iat>"
  Bus Selector2/8 -> Rate Transition9/1  "<TurboRackPos>"
  Bus Selector2/10 -> Rate Transition11/1  "<VarCompRatioPos>"
  Bus Selector2/3 -> Rate Transition4/1  "<Mat>"
  Unit Conversion/1 -> Rate Transition2/1
  Bus Selector2/14 -> Rate Transition15/1  "<IntkSwirlVlvPos>"
  Bus Selector2/7 -> Rate Transition8/1  "<ExhCamPhase>"
  Bus Selector2/6 -> Rate Transition7/1  "<IntkCamPhase>"
  CntrlRx/1 -> Bus Selector2/1
  Bus Selector2/11 -> Rate Transition12/1  "<IntkVlvLift>"
  Bus Selector2/20 -> Rate Transition21/1  "<EgrVlvDeltaPrs>"
  Bus Selector2/12 -> Rate Transition13/1  "<VarIntkRunLen>"
  Bus Selector2/5 -> Rate Transition6/1  "<WgAreaPct>"
  Bus Selector2/4 -> Rate Transition5/1  "<ThrPosPct>"
  Bus Selector/1 -> Rate Transition/1  "<EngTrqCmd>"
  Vcu/1 -> Bus Selector/1
  Brake/1 -> Bus Selector1/1
  Bus Selector1/1 -> Rate Transition1/1  "<ABSFlag>"
  Bus Selector2/22 -> Rate Transition23/1  "<AccelFdbk>"
  Rate Transition/1 -> TrqCmd/1  "TrqCmd"
  Rate Transition1/1 -> ABSFlag/1  "ABSFlag"
  Rate Transition2/1 -> EngSpd/1  "EngSpd"
  Rate Transition3/1 -> Map/1  "Map"
  Rate Transition4/1 -> Mat/1  "Mat"
  Rate Transition5/1 -> ThrPosPct/1  "ThrPosPct"
  Rate Transition6/1 -> WgAreaPct/1  "WgAreaPct"
  Rate Transition7/1 -> IntkCamPhase/1  "IntkCamPhase"
  Rate Transition8/1 -> ExhCamPhase/1  "ExhCamPhase"
  Rate Transition9/1 -> TurboRackPos/1  "TurboRackPos"
  Rate Transition10/1 -> EgrVlvAreaPct/1  "EgrVlvAreaPct"
  Rate Transition11/1 -> VarCompRatioPos/1  "VarCompRatioPos"
  Rate Transition12/1 -> IntkVlvLift/1  "IntkVlvLift"
  Rate Transition13/1 -> VarIntkRunLen/1  "VarIntkRunLen"
  Rate Transition14/1 -> Afr/1  "Afr"
  Rate Transition15/1 -> IntkSwirlVlvPos/1  "IntkSwirlVlvPos"
  Rate Transition16/1 -> TurboSpd/1  "TurboSpd"
  Rate Transition17/1 -> Baro/1  "Baro"
  Rate Transition18/1 -> IgSw/1  "IgSw"
  Rate Transition19/1 -> Iat/1  "Iat"
  Rate Transition20/1 -> Ect/1  "Ect"
  Rate Transition21/1 -> EgrVlvDeltaPrs/1  "EgrVlvDeltaPrs"
  Rate Transition22/1 -> EgrVlvInTemp/1  "EgrVlvInTemp"
  Rate Transition23/1 -> Accel/1  "Accel"
  Unit Conversion1/1 -> Rate Transition16/1

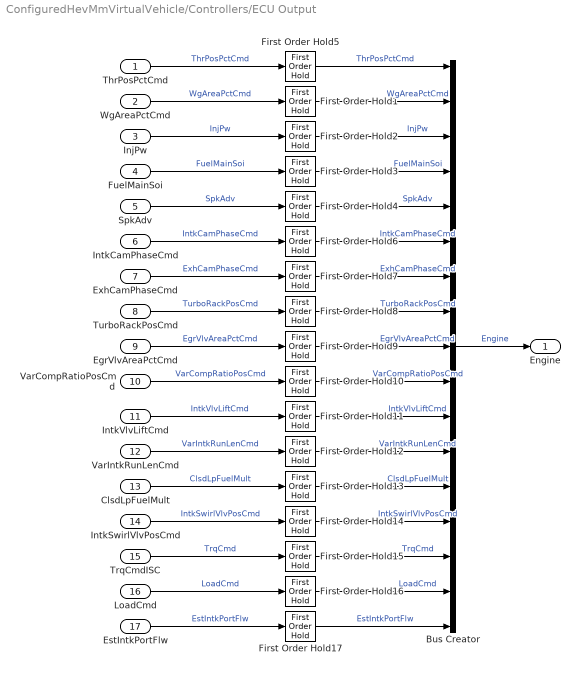
== system ConfiguredHevMmVirtualVehicle/Controllers/ECU Output ==
  ThrPosPctCmd : Inport
  WgAreaPctCmd : Inport  Port=2
  InjPw : Inport  Port=3
  FuelMainSoi : Inport  Port=4
  SpkAdv : Inport  Port=5
  IntkCamPhaseCmd : Inport  Port=6
  ExhCamPhaseCmd : Inport  Port=7
  TurboRackPosCmd : Inport  Port=8
  EgrVlvAreaPctCmd : Inport  Port=9
  VarCompRatioPosCmd : Inport  Port=10
  IntkVlvLiftCmd : Inport  Port=11
  VarIntkRunLenCmd : Inport  Port=12
  ClsdLpFuelMult : Inport  Port=13
  IntkSwirlVlvPosCmd : Inport  Port=14
  TrqCmdISC : Inport  Port=15
  LoadCmd : Inport  Port=16
  EstIntkPortFlw : Inport  Port=17
  Bus Creator : BusCreator  Inputs=17
  First Order Hold{1..17} (17 alike) : FirstOrderHold  ErrorTolerance=inf
  Engine : Outport
  wires:
  Bus Creator/1 -> Engine/1  "Engine"
  EstIntkPortFlw/1 -> First Order Hold17/1  "EstIntkPortFlw"
  ThrPosPctCmd/1 -> First Order Hold5/1  "ThrPosPctCmd"
  InjPw/1 -> First Order Hold2/1  "InjPw"
  SpkAdv/1 -> First Order Hold4/1  "SpkAdv"
  TrqCmdISC/1 -> First Order Hold15/1  "TrqCmd"
  VarCompRatioPosCmd/1 -> First Order Hold10/1  "VarCompRatioPosCmd"
  FuelMainSoi/1 -> First Order Hold3/1  "FuelMainSoi"
  IntkCamPhaseCmd/1 -> First Order Hold6/1  "IntkCamPhaseCmd"
  ClsdLpFuelMult/1 -> First Order Hold13/1  "ClsdLpFuelMult"
  WgAreaPctCmd/1 -> First Order Hold1/1  "WgAreaPctCmd"
  ExhCamPhaseCmd/1 -> First Order Hold7/1  "ExhCamPhaseCmd"
  TurboRackPosCmd/1 -> First Order Hold8/1  "TurboRackPosCmd"
  EgrVlvAreaPctCmd/1 -> First Order Hold9/1  "EgrVlvAreaPctCmd"
  IntkVlvLiftCmd/1 -> First Order Hold11/1  "IntkVlvLiftCmd"
  VarIntkRunLenCmd/1 -> First Order Hold12/1  "VarIntkRunLenCmd"
  IntkSwirlVlvPosCmd/1 -> First Order Hold14/1  "IntkSwirlVlvPosCmd"
  LoadCmd/1 -> First Order Hold16/1  "LoadCmd"
  First Order Hold5/1 -> Bus Creator/1  "ThrPosPctCmd"
  First Order Hold1/1 -> Bus Creator/2  "WgAreaPctCmd"
  First Order Hold2/1 -> Bus Creator/3  "InjPw"
  First Order Hold3/1 -> Bus Creator/4  "FuelMainSoi"
  First Order Hold4/1 -> Bus Creator/5  "SpkAdv"
  First Order Hold6/1 -> Bus Creator/6  "IntkCamPhaseCmd"
  First Order Hold7/1 -> Bus Creator/7  "ExhCamPhaseCmd"
  First Order Hold8/1 -> Bus Creator/8  "TurboRackPosCmd"
  First Order Hold9/1 -> Bus Creator/9  "EgrVlvAreaPctCmd"
  First Order Hold10/1 -> Bus Creator/10  "VarCompRatioPosCmd"
  First Order Hold11/1 -> Bus Creator/11  "IntkVlvLiftCmd"
  First Order Hold12/1 -> Bus Creator/12  "VarIntkRunLenCmd"
  First Order Hold13/1 -> Bus Creator/13  "ClsdLpFuelMult"
  First Order Hold14/1 -> Bus Creator/14  "IntkSwirlVlvPosCmd"
  First Order Hold15/1 -> Bus Creator/15  "TrqCmd"
  First Order Hold16/1 -> Bus Creator/16  "LoadCmd"
  First Order Hold17/1 -> Bus Creator/17  "EstIntkPortFlw"
